simulink model "LKA_Blender_TestBench"  (R2026b)
settings: Solver=ode4  StopTime=SCN.StopTime  FixedStep=0.005
undefined symbols (not defined in the file): LKA, ROAD, SCN, vehicle
settings Model: Creator=rithvin007  LastModifiedBy=rithvin007
settings DebuggingCC: AlgebraicLoopMsg=error

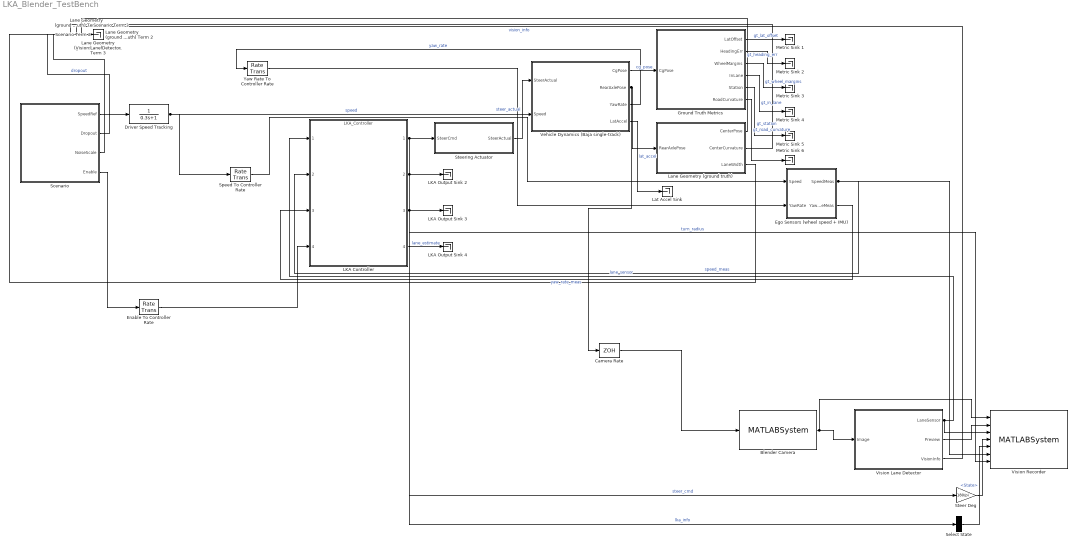
== system LKA_Blender_TestBench ==
  Blender Camera : MATLABSystem  System=LkaBlenderCamera  Vision=LKA.Vision  Ts=LKA.Ts  Host=127.0.0.1  Port=5560  FrameFile=/dev/shm/lka_blender_frame.jpg
      mask Type: LkaBlenderCamera
  Camera Rate : ZeroOrderHold  SampleTime=LKA.Ts
  Driver Speed Tracking : TransferFcn  Numerator=1  Denominator=[0.3 1]
  Ego Sensors (wheel speed + IMU) : Subsystem
  Enable To Controller Rate : RateTransition  OutPortSampleTime=LKA.Ts
  Ground Truth Metrics : Subsystem
  LKA Controller : ModelReference  ModelNameDialog=LKA_Controller  SimulationMode=Normal  ModelReferenceVersion=1.1
  LKA Output Sink 2 : Terminator
  LKA Output Sink 3 : Terminator
  LKA Output Sink 4 : Terminator
  Lane Geometry (ground truth) : Subsystem
  Lane Geometry (ground truth) Term 1 : Terminator
  Lane Geometry (ground truth) Term 2 : Terminator
  Lane Geometry (ground truth) Term 3 : Terminator
  Lat Accel Sink : Terminator
  Metric Sink {1..6} (6 alike) : Terminator
  Scenario : Subsystem
  Scenario Term 2 : Terminator
  Scenario Term 3 : Terminator
  Select State : BusSelector  OutputSignals=State
  Speed To Controller Rate : RateTransition  OutPortSampleTime=LKA.Ts
  Steer Deg : Gain  Gain=180/pi
  Steering Actuator : Subsystem
  Vehicle Dynamics (Baja single-track) : Subsystem
  Vision Lane Detector : Subsystem
  Vision Lane Detector Term 3 : Terminator
  Vision Recorder : MATLABSystem  System=LkaVisionRecorder  Vision=LKA.Vision  Ts=LKA.Ts
      mask Type: LkaVisionRecorder
  Yaw Rate To Controller Rate : RateTransition  OutPortSampleTime=LKA.Ts
  wires:
  Ground Truth Metrics/5(Station) -> Metric Sink 5/1  "gt_station"
  Ground Truth Metrics/4(InLane) -> Metric Sink 4/1  "gt_in_lane"
  Ground Truth Metrics/3(WheelMargins) -> Metric Sink 3/1  "gt_wheel_margins"
  Ground Truth Metrics/2(HeadingErr) -> Metric Sink 2/1  "gt_heading_err"
  Ground Truth Metrics/1(LatOffset) -> Metric Sink 1/1  "gt_lat_offset"
  Vehicle Dynamics (Baja single-track)/3(YawRate) -> Yaw Rate To Controller Rate/1  "yaw_rate"
  Ground Truth Metrics/6(RoadCurvature) -> Metric Sink 6/1  "gt_road_curvature"
  Vehicle Dynamics (Baja single-track)/2(RearAxlePose) -> Lane Geometry (ground truth)/1(RearAxlePose), Camera Rate/1
  Vehicle Dynamics (Baja single-track)/4(LatAccel) -> Lat Accel Sink/1  "lat_accel"
  LKA Controller/3 -> LKA Output Sink 3/1, Select State/1  "lka_info"
  Steering Actuator/1(SteerActual) -> Vehicle Dynamics (Baja single-track)/1(SteerActual)  "steer_actual"
  Driver Speed Tracking/1 -> Speed To Controller Rate/1, Vehicle Dynamics (Baja single-track)/2(Speed)  "speed"
  Enable To Controller Rate/1 -> LKA Controller/4
  Scenario/1(SpeedRef) -> Driver Speed Tracking/1
  Scenario/4(Enable) -> Enable To Controller Rate/1
  LKA Controller/1 -> Steering Actuator/1(SteerCmd), Steer Deg/1  "steer_cmd"
  Vehicle Dynamics (Baja single-track)/1(CgPose) -> Ground Truth Metrics/1(CgPose)  "cg_pose"
  LKA Controller/2 -> LKA Output Sink 2/1, Vision Recorder/7  "turn_radius"
  LKA Controller/4 -> LKA Output Sink 4/1  "lane_estimate"
  Lane Geometry (ground truth)/1(CenterPose) -> Lane Geometry (ground truth) Term 1/1
  Lane Geometry (ground truth)/2(CenterCurvature) -> Lane Geometry (ground truth) Term 2/1
  Lane Geometry (ground truth)/3(LaneWidth) -> Lane Geometry (ground truth) Term 3/1
  Scenario/2(Dropout) -> Scenario Term 2/1  "dropout"
  Scenario/3(NoiseScale) -> Scenario Term 3/1
  Camera Rate/1 -> Blender Camera/1
  Blender Camera/1 -> Vision Lane Detector/1(Image), Vision Recorder/1
  Vision Lane Detector/1(LaneSensor) -> LKA Controller/1, Vision Recorder/3  "lane_sensor"
  Speed To Controller Rate/1 -> Ego Sensors (wheel speed + IMU)/1(Speed)
  Yaw Rate To Controller Rate/1 -> Ego Sensors (wheel speed + IMU)/2(YawRate)
  Ego Sensors (wheel speed + IMU)/1(SpeedMeas) -> LKA Controller/2, Vision Recorder/6  "speed_meas"
  Ego Sensors (wheel speed + IMU)/2(YawRateMeas) -> LKA Controller/3  "yaw_rate_meas"
  Vision Lane Detector/2(Preview) -> Vision Recorder/2
  Steer Deg/1 -> Vision Recorder/4
  Select State/1 -> Vision Recorder/5  "<State>"
  Vision Lane Detector/3(VisionInfo) -> Vision Lane Detector Term 3/1  "vision_info"

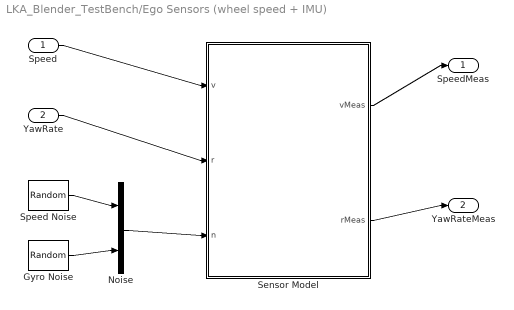
== system LKA_Blender_TestBench/Ego Sensors (wheel speed + IMU) ==
  Speed : Inport
  YawRate : Inport  Port=2
  Gyro Noise : RandomNumber  Seed=LKA.EgoSen.Seed(2)  SampleTime=LKA.Ts
  Noise : Mux  Inputs=2
  Sensor Model : MATLAB Function  TreatAsAtomicUnit=on
  Speed Noise : RandomNumber  Seed=LKA.EgoSen.Seed(1)  SampleTime=LKA.Ts
  SpeedMeas : Outport
  YawRateMeas : Outport  Port=2
  wires:
  Speed/1 -> Sensor Model/1(v)
  YawRate/1 -> Sensor Model/2(r)
  Speed Noise/1 -> Noise/1
  Gyro Noise/1 -> Noise/2
  Noise/1 -> Sensor Model/3(n)
  Sensor Model/1(vMeas) -> SpeedMeas/1
  Sensor Model/2(rMeas) -> YawRateMeas/1

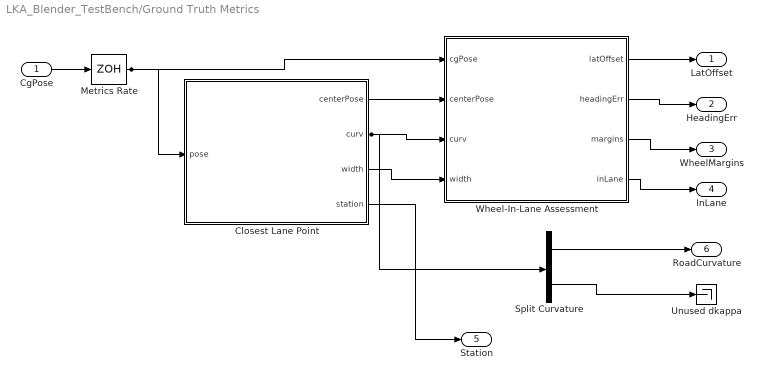
== system LKA_Blender_TestBench/Ground Truth Metrics ==
  CgPose : Inport
  Closest Lane Point : MATLAB Function  TreatAsAtomicUnit=on
  Metrics Rate : ZeroOrderHold  SampleTime=0.01
  Split Curvature : Demux  Outputs=2
  Unused dkappa : Terminator
  Wheel-In-Lane Assessment : MATLAB Function  TreatAsAtomicUnit=on
  LatOffset : Outport
  HeadingErr : Outport  Port=2
  WheelMargins : Outport  Port=3
  InLane : Outport  Port=4
  Station : Outport  Port=5
  RoadCurvature : Outport  Port=6
  wires:
  Wheel-In-Lane Assessment/4(inLane) -> InLane/1
  Wheel-In-Lane Assessment/3(margins) -> WheelMargins/1
  Wheel-In-Lane Assessment/2(headingErr) -> HeadingErr/1
  Split Curvature/1 -> RoadCurvature/1
  Closest Lane Point/4(station) -> Station/1
  Closest Lane Point/3(width) -> Wheel-In-Lane Assessment/4(width)
  Closest Lane Point/2(curv) -> Split Curvature/1, Wheel-In-Lane Assessment/3(curv)
  Wheel-In-Lane Assessment/1(latOffset) -> LatOffset/1
  Closest Lane Point/1(centerPose) -> Wheel-In-Lane Assessment/2(centerPose)
  Split Curvature/2 -> Unused dkappa/1
  Metrics Rate/1 -> Closest Lane Point/1(pose), Wheel-In-Lane Assessment/1(cgPose)
  CgPose/1 -> Metrics Rate/1

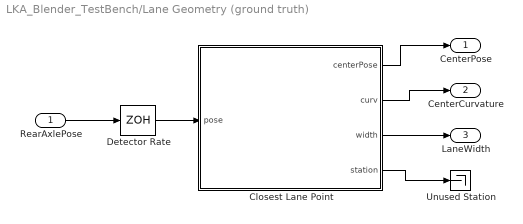
== system LKA_Blender_TestBench/Lane Geometry (ground truth) ==
  RearAxlePose : Inport
  Closest Lane Point : MATLAB Function  TreatAsAtomicUnit=on
  Detector Rate : ZeroOrderHold  SampleTime=LKA.Sen.Ts
  Unused Station : Terminator
  CenterPose : Outport
  CenterCurvature : Outport  Port=2
  LaneWidth : Outport  Port=3
  wires:
  Closest Lane Point/4(station) -> Unused Station/1
  Closest Lane Point/3(width) -> LaneWidth/1
  Closest Lane Point/2(curv) -> CenterCurvature/1
  Closest Lane Point/1(centerPose) -> CenterPose/1
  Detector Rate/1 -> Closest Lane Point/1(pose)
  RearAxlePose/1 -> Detector Rate/1

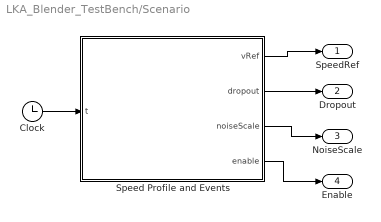
== system LKA_Blender_TestBench/Scenario ==
  Clock : Clock
  Speed Profile and Events : MATLAB Function  TreatAsAtomicUnit=on
  SpeedRef : Outport
  Dropout : Outport  Port=2
  NoiseScale : Outport  Port=3
  Enable : Outport  Port=4
  wires:
  Speed Profile and Events/4(enable) -> Enable/1
  Speed Profile and Events/3(noiseScale) -> NoiseScale/1
  Speed Profile and Events/2(dropout) -> Dropout/1
  Speed Profile and Events/1(vRef) -> SpeedRef/1
  Clock/1 -> Speed Profile and Events/1(t)

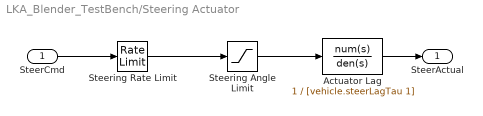
== system LKA_Blender_TestBench/Steering Actuator ==
  SteerCmd : Inport
  Actuator Lag : TransferFcn  Numerator=1  Denominator=[vehicle.steerLagTau 1]
  Steering Angle Limit : Saturate  UpperLimit=vehicle.maxSteerAngle  LowerLimit=-vehicle.maxSteerAngle
  Steering Rate Limit : RateLimiter  RisingSlewLimit=vehicle.maxSteerRate  FallingSlewLimit=-vehicle.maxSteerRate  SampleTimeMode=inherited
  SteerActual : Outport
  wires:
  Actuator Lag/1 -> SteerActual/1
  Steering Angle Limit/1 -> Actuator Lag/1
  Steering Rate Limit/1 -> Steering Angle Limit/1
  SteerCmd/1 -> Steering Rate Limit/1

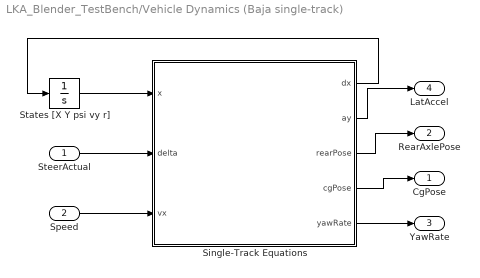
== system LKA_Blender_TestBench/Vehicle Dynamics (Baja single-track) ==
  SteerActual : Inport
  Speed : Inport  Port=2
  Single-Track Equations : MATLAB Function  TreatAsAtomicUnit=on
  States [X Y psi vy r] : Integrator  InitialCondition=SCN.X0
  CgPose : Outport
  RearAxlePose : Outport  Port=2
  YawRate : Outport  Port=3
  LatAccel : Outport  Port=4
  wires:
  Single-Track Equations/4(cgPose) -> CgPose/1
  Single-Track Equations/3(rearPose) -> RearAxlePose/1
  Single-Track Equations/5(yawRate) -> YawRate/1
  Single-Track Equations/2(ay) -> LatAccel/1
  Single-Track Equations/1(dx) -> States [X Y psi vy r]/1
  Speed/1 -> Single-Track Equations/3(vx)
  SteerActual/1 -> Single-Track Equations/2(delta)
  States [X Y psi vy r]/1 -> Single-Track Equations/1(x)

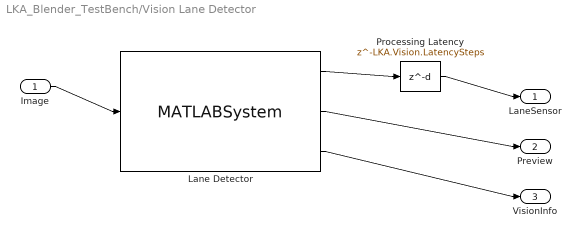
== system LKA_Blender_TestBench/Vision Lane Detector ==
  Image : Inport
  Lane Detector : MATLABSystem  System=LkaVisionLaneDetector  Vision=LKA.Vision  Ts=LKA.Ts
      mask Type: LkaVisionLaneDetector
  Processing Latency : Delay  DelayLength=LKA.Vision.LatencySteps  InitialCondition=0  SampleTime=LKA.Ts
  LaneSensor : Outport  OutDataTypeStr=Bus: LaneSensorBus
  Preview : Outport  Port=2
  VisionInfo : Outport  Port=3
  wires:
  Image/1 -> Lane Detector/1
  Lane Detector/1 -> Processing Latency/1
  Processing Latency/1 -> LaneSensor/1
  Lane Detector/2 -> Preview/1
  Lane Detector/3 -> VisionInfo/1

== matlab function LKA_Blender_TestBench/Vehicle Dynamics (Baja single-track)/Single-Track Equations ==
  data: x input; dx output; delta input; vx input; ay output; rearPose output; cgPose output; yawRate output; vehicle parameter
function [dx, ay, rearPose, cgPose, yawRate] = fcn(x, delta, vx, vehicle)
% Nonlinear bicycle model with saturating tyres (see lka_single_track_dynamics.m)
[dx, ay, rearPose] = lka_single_track_dynamics(x, delta, vx, vehicle);
cgPose = [x(1) x(2) x(3)];
yawRate = x(5);

== matlab function LKA_Blender_TestBench/Scenario/Speed Profile and Events ==
  data: t input; vRef output; dropout output; noiseScale output; enable output; SCN parameter
function [vRef, dropout, noiseScale, enable] = fcn(t, SCN)
% Driver speed profile v = min(V0 + a*t, VSet) and forced detector outages
vRef = min(SCN.V0 + SCN.Accel*t, SCN.VSet);
dropout = [0; 0];
for k = 1:size(SCN.Dropouts, 1)
    if t >= SCN.Dropouts(k,1) && t < SCN.Dropouts(k,2)
        side = SCN.Dropouts(k,3);
        if side == 1 || side == 3, dropout(1) = 1; end
        if side == 2 || side == 3, dropout(2) = 1; end
    end
end
noiseScale = SCN.NoiseScale;
enable = true;

== matlab function LKA_Blender_TestBench/Lane Geometry (ground truth)/Closest Lane Point ==
  data: pose input; centerPose output; curv output; width output; station output; ROAD parameter
function [centerPose, curv, width, station] = fcn(pose, ROAD)
% Foot point of the pose on the true lane centreline (windowed search, see lka_road_closest_point.m)
persistent idx
if isempty(idx), idx = 0; end
[centerPose, curv, width, station, idx] = lka_road_closest_point(pose(1), pose(2), idx, ...
    ROAD.s, ROAD.x, ROAD.y, ROAD.psi, ROAD.kappa, ROAD.dkappa, ROAD.width);

== matlab function LKA_Blender_TestBench/Ego Sensors (wheel speed + IMU)/Sensor Model ==
  data: v input; vMeas output; r input; n input; rMeas output; LKA parameter
function [vMeas, rMeas] = fcn(v, r, n, LKA)
% Wheel-speed sensor and gyro with scale error, bias and noise (lka_ego_sensor_model.m)
[vMeas, rMeas] = lka_ego_sensor_model(v, r, n, LKA.EgoSen);

== matlab function LKA_Blender_TestBench/Ground Truth Metrics/Closest Lane Point ==
  data: pose input; centerPose output; curv output; width output; station output; ROAD parameter
function [centerPose, curv, width, station] = fcn(pose, ROAD)
% Foot point of the pose on the true lane centreline (windowed search, see lka_road_closest_point.m)
persistent idx
if isempty(idx), idx = 0; end
[centerPose, curv, width, station, idx] = lka_road_closest_point(pose(1), pose(2), idx, ...
    ROAD.s, ROAD.x, ROAD.y, ROAD.psi, ROAD.kappa, ROAD.dkappa, ROAD.width);

== matlab function LKA_Blender_TestBench/Ground Truth Metrics/Wheel-In-Lane Assessment ==
  data: cgPose input; latOffset output; centerPose input; curv input; width input; headingErr output; margins output; inLane output; ROAD parameter; vehicle parameter
function [latOffset, headingErr, margins, inLane] = fcn(cgPose, centerPose, curv, width, ROAD, vehicle)
% True CG offset, heading error and tyre-edge-to-line margins (rulebook K.2.4)
[latOffset, headingErr, margins, inLane] = lka_ground_truth_metrics(cgPose, centerPose, curv, width, ROAD.lineWidth, vehicle);
